simulink library "controls_element_lib"  (R2018b)
settings: Solver=VariableStepAuto  StartTime=0.0  StopTime=10.0  RelTol=1e-3
undefined symbols (not defined in the file): F_NOM, I_INV_BASE, j, P_INV_NOM, S_INV_NOM, S_NOM, S_PLANT, VHV_NOM, VLL_INV_NOM, VLL_NOM, Z_INV_BASE
libraries: simulink x20, $bdroot x5
(part 1 of 2)
settings Model: Creator=HussamAlatrash  LastModifiedBy=ahhei
settings DataIOCC: ReturnWorkspaceOutputs=on
settings DebuggingCC: UnconnectedInputMsg=none  UnconnectedOutputMsg=none  UnconnectedLineMsg=none
settings ModelReferenceCC: EnableRefExpFcnMdlSchedulingChecks=off
settings RTWCC: Description=Generic Real-Time Target
settings ConfigComp: CovBoundaryAbsTol=1.0e-5

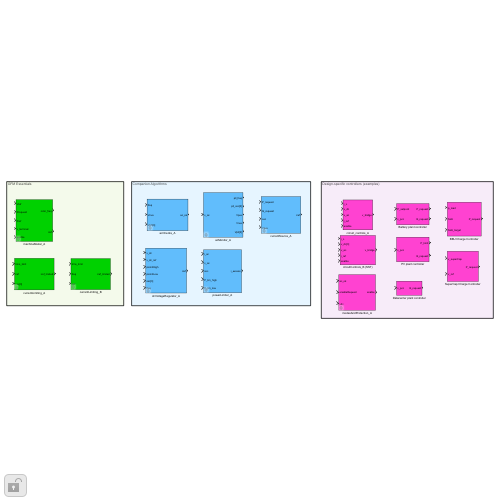
[thumbnail: Simulink's stored preview of the top-level diagram]
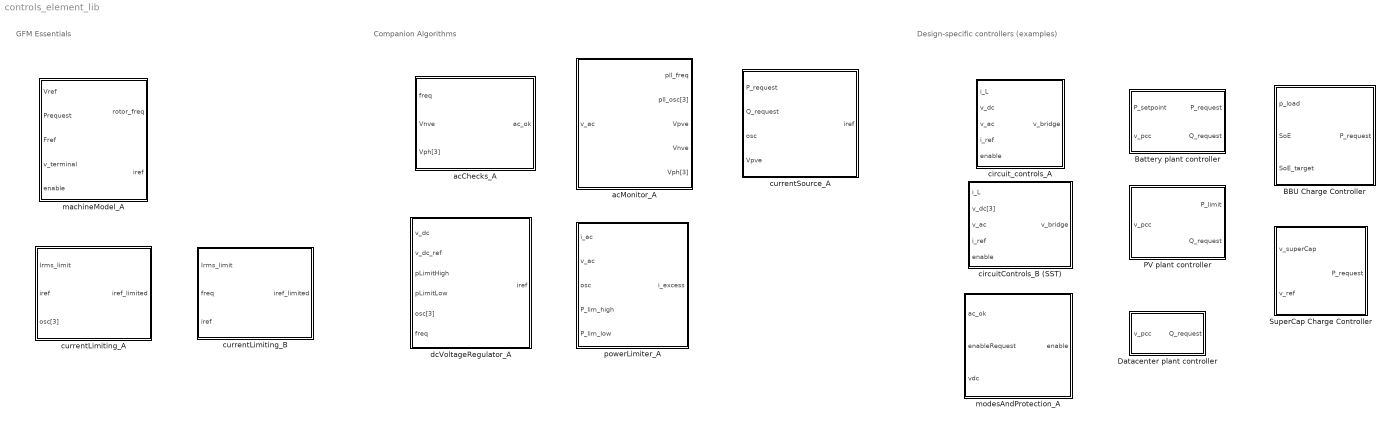
== system controls_element_lib ==
  note: Design-specific controllers (examples)
  note: Companion Algorithms
  note: GFM Essentials
  BBU Charge Controller : Subsystem
  Battery plant controller : Subsystem
  Datacenter plant controller : Subsystem
  PV plant controller : Subsystem
  SuperCap Charge Controller : Subsystem
  acChecks_A : Subsystem  mask{VllRated=VLL_NOM, nominalFrequency=F_NOM, tRequalify=2, T_CNTL=1e-3}
      mask prompts: VllRated "Rated line-to-line voltage (V)"; nominalFrequency "Nominal line frequency (Hz)"; tRequalify "Reconnection time (sec)"; T_CNTL "Operating sample time"
  acMonitor_A : Subsystem  mask{VllRated=VLL_NOM, nominalFrequency=F_NOM}
      mask prompts: VllRated "Rated line-to-line voltage (V)"; nominalFrequency "Nominal line frequency (Hz)"
  circuitControls_B (SST) : Subsystem
  circuit_controls_A : Subsystem
  currentLimiting_A : Subsystem  mask{IRated=I_INV_BASE, peakSoftLimit=2.6, peakHardLimit=3.6}
      mask prompts: IRated "Rated current (A)"; peakSoftLimit "Soft peak limit (pu)"; peakHardLimit "Hard peak limit (pu)"
  currentLimiting_B : Subsystem  mask{IRated=I_INV_BASE, peakSoftLimit=2.6, peakHardLimit=3.6}
      mask prompts: IRated "Rated current (A)"; peakSoftLimit "Soft peak limit (pu)"; peakHardLimit "Hard peak limit (pu)"
  currentSource_A : Subsystem  mask{VllRated=VLL_NOM, SRated=S_NOM, nominalFrequency=F_NOM, Plimit=1, Qlimit=0.43}
      mask prompts: VllRated "Rated line-to-line voltage (V)"; SRated "Rated power (VA)"; nominalFrequency "Nominal line frequency (Hz)"; Plimit "Real power request limit (pu)"; Qlimit "Reactive power request limit (pu)"
  dcVoltageRegulator_A : Subsystem  mask{kp=20e3, kSlowPath=0, wSlowPath=5, pLimitExternalMinimum=0.05*S_NOM, vdc_deadband=0, VllRated=VLL_INV_NOM}
      mask prompts: kp "Proportional gain (W/V)"; kSlowPath "Slow path gain (W/V)"; wSlowPath "Slow path bandwidth (rad)"; pLimitExternalMinimum "Minimum value for external power limit (W)"; vdc_deadband "Deadband around reference voltage (V)"; VllRated "Rated Voltage (Volts, line-to-line)"
  machineModel_A : Subsystem  mask{SRated=S_INV_NOM, VllRated=VLL_INV_NOM, nominalFrequency=F_NOM, inertialConstant=2.5, kDroop=1, kDamper=2, Xs=0.3, rs=0.08, Qlimit=0.5, wExciter=10}
      mask prompts: SRated "Rated power (VA)"; VllRated "Rated Voltage (Volts, line-to-line)"; nominalFrequency "Nominal frequency (Hz)"; inertialConstant "Inertial constant (seconds)"; kDroop "Droop gain (pu/Hz)"; kDamper "Damper gain (pu/Hz)"; Xs "Stator reactance (pu)"; rs "Stator resistance (pu)"; Qlimit "Reactive power request limit (pu)"; wExciter "Exciter Bandwidth (rad)"
  modesAndProtection_A : Subsystem  mask{dcOvervotlageThreshold=1800, dcUndervotlageThreshold=700, dcTripClearTimeout=0.2}
      mask prompts: dcOvervotlageThreshold "Dc overvoltage threshold"; dcUndervotlageThreshold "Dc undervoltage threshold"; dcTripClearTimeout "Dc protection clear time"
  powerLimiter_A : Subsystem  mask{VllRated=VLL_NOM, nominalFrequency=F_NOM, wPowerLimiter=3}
      mask prompts: VllRated "Rated line-to-line voltage (V)"; nominalFrequency "Nominal line frequency (Hz)"; wPowerLimiter "Bandwidth (rad)"

== system controls_element_lib/BBU Charge Controller ==
  p_load : Inport
  SoE : Inport  Port=2
  SoE_target : Inport  Port=3
  Gain : Gain  Gain=-1
  Gain4 : Gain  Gain=1e6/0.25
  Saturation1 : Saturate  UpperLimit=P_INV_NOM  LowerLimit=-P_INV_NOM
  Sum2 : Sum  Inputs=++|
  Sum3 : Sum  Inputs=|+-
  Transfer Fcn : TransferFcn  Denominator=[0.2 1]
  Transfer Fcn1 : TransferFcn  Denominator=[5 1]
  P_request : Outport
  wires:
  SoE/1 -> Sum3/1
  Gain/1 -> Transfer Fcn1/1
  Saturation1/1 -> Sum2/2  "P_charge_control"
  Sum3/1 -> Transfer Fcn/1
  SoE_target/1 -> Sum3/2
  Transfer Fcn1/1 -> Sum2/1  "P_dc"
  Gain4/1 -> Saturation1/1
  Sum2/1 -> P_request/1
  p_load/1 -> Gain/1
  Transfer Fcn/1 -> Gain4/1

== system controls_element_lib/Battery plant controller ==
  P_setpoint : Inport
  v_pcc : Inport  Port=2
  Gain : Gain  Gain=-1
  Gain1 : Gain  Gain=S_PLANT
  Gain2 : Gain  Gain=S_PLANT
  Gain4 : Gain  Gain=1/VHV_NOM
  LVRT_foldback : Subsystem
  Meter : Subsystem
  Saturation : Saturate  UpperLimit=0.9*S_PLANT  LowerLimit=-0.9*S_PLANT
  Saturation Dynamic : simulink/Discontinuities/Saturation Dynamic  OutMin=[]  OutMax=[]  OutDataTypeStr=Inherit: Same as second input  OutDataType=fixdt(1, 16)  OutScaling=2^-10  DoSatur=off
  VoltVAr : Subsystem
  P_request : Outport
  Q_request : Outport  Port=2
  wires:
  VoltVAr/1(Q) -> Gain1/1
  Meter/1(V_estimate) -> LVRT_foldback/1(Vpve_pu), VoltVAr/1(V)  "V_pu_plant"
  Gain1/1 -> Q_request/1  "Q_request"
  v_pcc/1 -> Gain4/1
  P_setpoint/1 -> Saturation/1
  Gain4/1 -> Meter/1(v)
  Saturation/1 -> Saturation Dynamic/2
  Gain2/1 -> Gain/1, Saturation Dynamic/1
  LVRT_foldback/1(limit_pu) -> Gain2/1  "spinout_limit_Vpcc"
  Saturation Dynamic/1 -> P_request/1  "P_request"
  Gain/1 -> Saturation Dynamic/3

== system controls_element_lib/Datacenter plant controller ==
  v_pcc : Inport
  Gain4 : Gain  Gain=1/VLL_INV_NOM
  Meter : Subsystem
  SRated2 : Gain  Gain=S_PLANT
  VoltVAr : Subsystem
  Q_request : Outport
  wires:
  VoltVAr/1(Q) -> SRated2/1
  Gain4/1 -> Meter/1(v)
  Meter/1(V_estimate) -> VoltVAr/1(V)  "V_pu_plant"
  SRated2/1 -> Q_request/1  "Q_request"
  v_pcc/1 -> Gain4/1

== system controls_element_lib/PV plant controller ==
  v_pcc : Inport
  Frequency foldback : Subsystem
  Gain1 : Gain  Gain=S_PLANT
  Gain2 : Gain  Gain=S_PLANT
  Gain4 : Gain  Gain=1/VHV_NOM
  Meter : Subsystem
  VoltVAr : Subsystem
  P_limit : Outport
  Q_request : Outport  Port=2
  wires:
  VoltVAr/1(Q) -> Gain1/1
  Gain4/1 -> Meter/1(v)
  Meter/2(V_estimate) -> VoltVAr/1(V)  "V_pu_plant"
  Gain1/1 -> Q_request/1  "Q_request"
  v_pcc/1 -> Gain4/1
  Meter/1(f) -> Frequency foldback/1(f)
  Frequency foldback/1(limit_pu) -> Gain2/1
  Gain2/1 -> P_limit/1  "P_limit"

== system controls_element_lib/SuperCap Charge Controller ==
  v_superCap : Inport
  v_ref : Inport  Port=2
  Gain4 : Gain  Gain=S_INV_NOM/100
  Saturation1 : Saturate  UpperLimit=S_INV_NOM  LowerLimit=-S_INV_NOM
  Sum3 : Sum  Inputs=|+-
  P_request : Outport
  wires:
  Saturation1/1 -> P_request/1
  v_ref/1 -> Sum3/2
  Sum3/1 -> Gain4/1
  v_superCap/1 -> Sum3/1
  Gain4/1 -> Saturation1/1

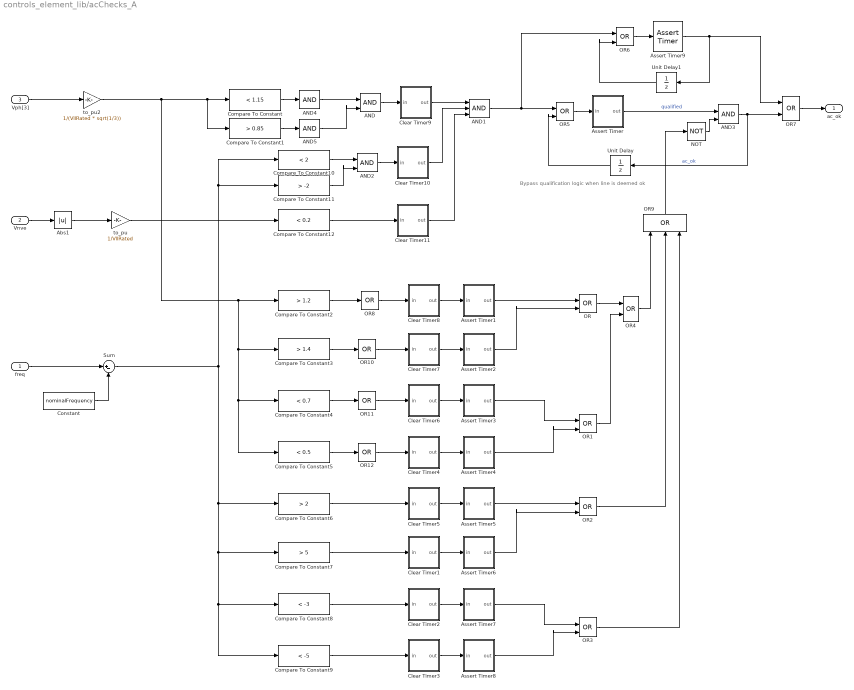
== system controls_element_lib/acChecks_A ==
  note: Bypass qualification logic when line is deemed ok
  freq : Inport
  Vnve : Inport  Port=2
  Vph[3] : Inport  Port=3
  AND : Logic  IconShape=distinctive  AllPortsSameDT=off  OutDataTypeStr=boolean
  AND1 : Logic  Inputs=3  IconShape=distinctive  AllPortsSameDT=off  OutDataTypeStr=boolean
  AND2 : Logic  IconShape=distinctive  AllPortsSameDT=off  OutDataTypeStr=boolean
  AND3 : Logic  IconShape=distinctive  AllPortsSameDT=off  OutDataTypeStr=boolean
  AND4 : Logic  Inputs=1  IconShape=distinctive  AllPortsSameDT=off  OutDataTypeStr=boolean
  AND5 : Logic  Inputs=1  IconShape=distinctive  AllPortsSameDT=off  OutDataTypeStr=boolean
  Abs1 : Abs
  Assert Timer : Subsystem  mask{T_STEP=T_CNTL, TIMEOUT=300}
      mask prompts: T_STEP "Time step"
  Assert Timer1 : Subsystem  mask{T_STEP=T_CNTL, TIMEOUT=60}
      mask prompts: T_STEP "Time step"
  Assert Timer2 : Subsystem  mask{T_STEP=T_CNTL, TIMEOUT=10}
      mask prompts: T_STEP "Time step"
  Assert Timer3 : Subsystem  mask{T_STEP=T_CNTL, TIMEOUT=60}
      mask prompts: T_STEP "Time step"
  Assert Timer4 : Subsystem  mask{T_STEP=T_CNTL, TIMEOUT=10}
      mask prompts: T_STEP "Time step"
  Assert Timer5 : Subsystem  mask{T_STEP=T_CNTL, TIMEOUT=60}
      mask prompts: T_STEP "Time step"
  Assert Timer6 : Subsystem  mask{T_STEP=T_CNTL, TIMEOUT=10}
      mask prompts: T_STEP "Time step"
  Assert Timer7 : Subsystem  mask{T_STEP=T_CNTL, TIMEOUT=60}
      mask prompts: T_STEP "Time step"
  Assert Timer8 : Subsystem  mask{T_STEP=T_CNTL, TIMEOUT=10}
      mask prompts: T_STEP "Time step"
  Assert Timer9 : $bdroot/acChecks_A/Assert Timer  T_STEP=T_CNTL  TIMEOUT=tRequalify
  Clear Timer1 : Subsystem  mask{T_STEP=T_CNTL, TIMEOUT=0.1, TIMER_INIT=0.1}
      mask prompts: T_STEP "Time step"; TIMER_INIT "Timer initial value"
  Clear Timer10 : Subsystem  mask{T_STEP=T_CNTL, TIMEOUT=0.1, TIMER_INIT=0}
      mask prompts: T_STEP "Time step"; TIMER_INIT "Timer initial value"
  Clear Timer11 : Subsystem  mask{T_STEP=T_CNTL, TIMEOUT=0.1, TIMER_INIT=0}
      mask prompts: T_STEP "Time step"; TIMER_INIT "Timer initial value"
  Clear Timer2 : Subsystem  mask{T_STEP=T_CNTL, TIMEOUT=0.1, TIMER_INIT=0.1}
      mask prompts: T_STEP "Time step"; TIMER_INIT "Timer initial value"
  Clear Timer3 : Subsystem  mask{T_STEP=T_CNTL, TIMEOUT=0.1, TIMER_INIT=0.1}
      mask prompts: T_STEP "Time step"; TIMER_INIT "Timer initial value"
  Clear Timer4 : Subsystem  mask{T_STEP=T_CNTL, TIMEOUT=0.1, TIMER_INIT=0}
      mask prompts: T_STEP "Time step"; TIMER_INIT "Timer initial value"
  Clear Timer5 : Subsystem  mask{T_STEP=T_CNTL, TIMEOUT=0.1, TIMER_INIT=0.1}
      mask prompts: T_STEP "Time step"; TIMER_INIT "Timer initial value"
  Clear Timer6 : Subsystem  mask{T_STEP=T_CNTL, TIMEOUT=0.1, TIMER_INIT=0}
      mask prompts: T_STEP "Time step"; TIMER_INIT "Timer initial value"
  Clear Timer7 : Subsystem  mask{T_STEP=T_CNTL, TIMEOUT=0.1, TIMER_INIT=0}
      mask prompts: T_STEP "Time step"; TIMER_INIT "Timer initial value"
  Clear Timer8 : Subsystem  mask{T_STEP=T_CNTL, TIMEOUT=0.1, TIMER_INIT=0}
      mask prompts: T_STEP "Time step"; TIMER_INIT "Timer initial value"
  Clear Timer9 : Subsystem  mask{T_STEP=T_CNTL, TIMEOUT=0.1, TIMER_INIT=0}
      mask prompts: T_STEP "Time step"; TIMER_INIT "Timer initial value"
  Compare To Constant : simulink/Logic and Bit Operations/Compare To Constant  relop=<  const=1.15  OutDataTypeStr=boolean
  Compare To Constant1 : simulink/Logic and Bit Operations/Compare To Constant  relop=>  const=0.85  OutDataTypeStr=boolean
  Compare To Constant10 : simulink/Logic and Bit Operations/Compare To Constant  relop=<  const=2  OutDataTypeStr=boolean
  Compare To Constant11 : simulink/Logic and Bit Operations/Compare To Constant  relop=>  const=-2  OutDataTypeStr=boolean
  Compare To Constant12 : simulink/Logic and Bit Operations/Compare To Constant  relop=<  const=0.2  OutDataTypeStr=boolean
  Compare To Constant2 : simulink/Logic and Bit Operations/Compare To Constant  relop=>  const=1.2  OutDataTypeStr=boolean
  Compare To Constant3 : simulink/Logic and Bit Operations/Compare To Constant  relop=>  const=1.4  OutDataTypeStr=boolean
  Compare To Constant4 : simulink/Logic and Bit Operations/Compare To Constant  relop=<  const=0.7  OutDataTypeStr=boolean
  Compare To Constant5 : simulink/Logic and Bit Operations/Compare To Constant  relop=<  const=0.5  OutDataTypeStr=boolean
  Compare To Constant6 : simulink/Logic and Bit Operations/Compare To Constant  relop=>  const=2  OutDataTypeStr=boolean
  Compare To Constant7 : simulink/Logic and Bit Operations/Compare To Constant  relop=>  const=5  OutDataTypeStr=boolean
  Compare To Constant8 : simulink/Logic and Bit Operations/Compare To Constant  relop=<  const=-3  OutDataTypeStr=boolean
  Compare To Constant9 : simulink/Logic and Bit Operations/Compare To Constant  relop=<  const=-5  OutDataTypeStr=boolean
  Constant : Constant  Value=nominalFrequency
  NOT : Logic  Operator=NOT  IconShape=distinctive  AllPortsSameDT=off  OutDataTypeStr=boolean
  OR{,1..7} (8 alike) : Logic  Operator=OR  IconShape=distinctive  AllPortsSameDT=off  OutDataTypeStr=boolean
  OR{8,10..12} (4 alike) : Logic  Operator=OR  Inputs=1  IconShape=distinctive  AllPortsSameDT=off  OutDataTypeStr=boolean
  OR9 : Logic  Operator=OR  Inputs=3  IconShape=distinctive  AllPortsSameDT=off  OutDataTypeStr=boolean
  Sum : Sum  Inputs=|+-
  Unit Delay : UnitDelay  SampleTime=T_CNTL  HasFrameUpgradeWarning=on
  Unit Delay1 : UnitDelay  SampleTime=T_CNTL  HasFrameUpgradeWarning=on
  to_pu : Gain  Gain=1/VllRated
  to_pu2 : Gain  Gain=1/(VllRated * sqrt(1/3))
  ac_ok : Outport
  wires:
  AND5/1 -> AND/2
  AND4/1 -> AND/1
  AND/1 -> Clear Timer9/1(in)
  OR12/1 -> Clear Timer4/1(in)
  OR11/1 -> Clear Timer6/1(in)
  OR10/1 -> Clear Timer7/1(in)
  OR8/1 -> Clear Timer8/1(in)
  OR2/1 -> OR9/2
  AND3/1 -> OR7/2, Unit Delay/1  "ac_ok"
  Clear Timer4/1(out) -> Assert Timer4/1(in)
  OR/1 -> OR4/1
  Clear Timer9/1(out) -> AND1/1
  Compare To Constant10/1 -> AND2/1
  Assert Timer2/1(out) -> OR/2
  Sum/1 -> Compare To Constant9/1, Compare To Constant8/1, Compare To Constant7/1, Compare To Constant6/1, Compare To Constant10/1, Compare To Constant11/1
  Clear Timer7/1(out) -> Assert Timer2/1(in)
  Clear Timer3/1(out) -> Assert Timer8/1(in)
  Clear Timer10/1(out) -> AND1/2
  Compare To Constant7/1 -> Clear Timer1/1(in)
  Compare To Constant5/1 -> OR12/1
  Clear Timer2/1(out) -> Assert Timer7/1(in)
  OR1/1 -> OR4/2
  Compare To Constant8/1 -> Clear Timer2/1(in)
  AND1/1 -> OR5/1, OR6/1
  Clear Timer6/1(out) -> Assert Timer3/1(in)
  Assert Timer6/1(out) -> OR2/2
  Compare To Constant4/1 -> OR11/1
  Compare To Constant11/1 -> AND2/2
  Compare To Constant9/1 -> Clear Timer3/1(in)
  AND2/1 -> Clear Timer10/1(in)
  Compare To Constant3/1 -> OR10/1
  Compare To Constant/1 -> AND4/1
  Assert Timer3/1(out) -> OR1/1
  NOT/1 -> AND3/2
  Vnve/1 -> Abs1/1
  Assert Timer8/1(out) -> OR3/2
  Assert Timer7/1(out) -> OR3/1
  Clear Timer8/1(out) -> Assert Timer1/1(in)
  Clear Timer1/1(out) -> Assert Timer6/1(in)
  Compare To Constant6/1 -> Clear Timer5/1(in)
  Clear Timer5/1(out) -> Assert Timer5/1(in)
  Assert Timer5/1(out) -> OR2/1
  Assert Timer4/1(out) -> OR1/2
  OR3/1 -> OR9/3
  Assert Timer/1(out) -> AND3/1  "qualified"
  Compare To Constant1/1 -> AND5/1
  Compare To Constant2/1 -> OR8/1
  OR5/1 -> Assert Timer/1(in)
  Clear Timer11/1(out) -> AND1/3
  Compare To Constant12/1 -> Clear Timer11/1(in)
  Assert Timer1/1(out) -> OR/1
  Unit Delay/1 -> OR5/2
  Abs1/1 -> to_pu/1
  to_pu2/1 -> Compare To Constant3/1, Compare To Constant4/1, Compare To Constant5/1, Compare To Constant2/1, Compare To Constant1/1, Compare To Constant/1
  to_pu/1 -> Compare To Constant12/1
  freq/1 -> Sum/1
  Constant/1 -> Sum/2
  Unit Delay1/1 -> OR6/2
  OR6/1 -> Assert Timer9/1
  Assert Timer9/1 -> OR7/1, Unit Delay1/1
  OR7/1 -> ac_ok/1
  OR9/1 -> NOT/1
  OR4/1 -> OR9/1
  Vph[3]/1 -> to_pu2/1

== system controls_element_lib/acMonitor_A ==
  v_ac : Inport
  Analyzer_V : Subsystem
  Gain2 : Gain  Gain=2
  PLL_3ph : Subsystem
  RMS_Analyzer : Subsystem
  SOGI : Subsystem
  to_pu : Gain  Gain=1/VllRated
  pll_freq : Outport
  pll_osc[3] : Outport  Port=2
  Vpve : Outport  Port=3
  Vnve : Outport  Port=4
  Vph[3] : Outport  Port=5
  wires:
  to_pu/1 -> PLL_3ph/1(ref)
  v_ac/1 -> RMS_Analyzer/1(in), Analyzer_V/1(in[3]), to_pu/1
  PLL_3ph/2(freq) -> pll_freq/1, Gain2/1
  PLL_3ph/1(osc[3]) -> Analyzer_V/2(osc[3]), pll_osc[3]/1
  Analyzer_V/3(Pve) -> Vpve/1
  Analyzer_V/4(Nve) -> Vnve/1
  RMS_Analyzer/1(RMS) -> SOGI/1(in)
  Gain2/1 -> SOGI/2(fnom)
  SOGI/1(notch) -> Vph[3]/1

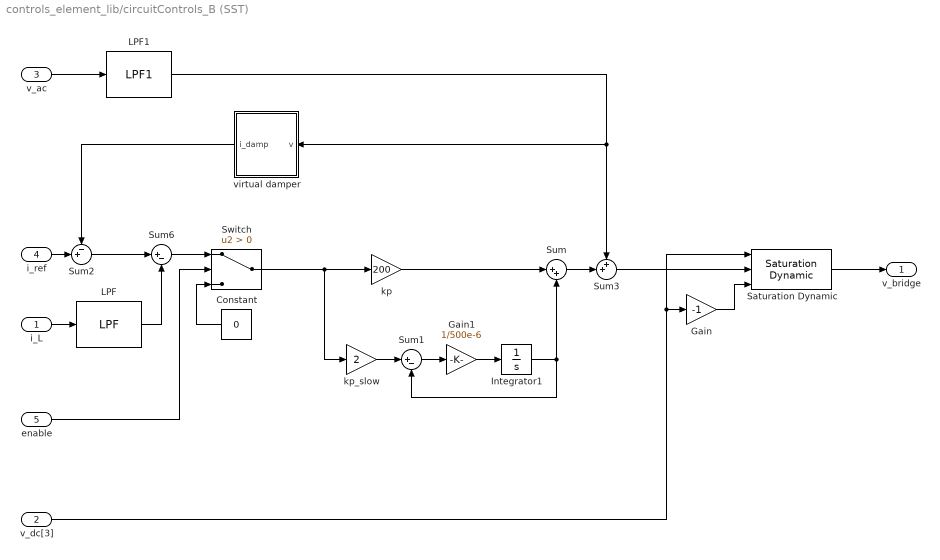
== system controls_element_lib/circuitControls_B (SST) ==
  i_L : Inport
  v_dc[3] : Inport  Port=2
  v_ac : Inport  Port=3
  i_ref : Inport  Port=4
  enable : Inport  Port=5
  Constant : Constant  Value=0
  Gain : Gain  Gain=-1
  Gain1 : Gain  Gain=1/500e-6
  Integrator1 : Integrator
  LPF : $bdroot/circuit_controls_A/LPF  SystemSampleTime=-1  EmptyChoice=off  PassThrough=off  PassThroughVariantControl=(default)  EmptyChoiceVariantControl=(default)  Latency=0  AutoFrameSizeCalculation=off
  LPF1 : $bdroot/circuit_controls_A/LPF1  SystemSampleTime=-1  EmptyChoice=off  PassThrough=off  PassThroughVariantControl=(default)  EmptyChoiceVariantControl=(default)  Latency=0  AutoFrameSizeCalculation=off
  Saturation Dynamic : simulink/Discontinuities/Saturation Dynamic  OutMin=[]  OutMax=[]  OutDataTypeStr=Inherit: Same as second input  OutDataType=fixdt(1, 16)  OutScaling=2^-10  DoSatur=off
  Sum : Sum  Inputs=|++
  Sum1 : Sum  Inputs=|+-
  Sum2 : Sum  Inputs=-+|
  Sum3 : Sum  Inputs=++|
  Sum6 : Sum  Inputs=|+-
  Switch : Switch  Criteria=u2 > Threshold
  kp : Gain  Gain=200
  kp_slow : Gain  Gain=2
  virtual damper : Subsystem
  v_bridge : Outport
  wires:
  Gain/1 -> Saturation Dynamic/3
  kp_slow/1 -> Sum1/1
  Gain1/1 -> Integrator1/1
  Sum1/1 -> Gain1/1
  Integrator1/1 -> Sum1/2, Sum/2
  kp/1 -> Sum/1
  Sum2/1 -> Sum6/1
  Saturation Dynamic/1 -> v_bridge/1
  i_L/1 -> LPF/1
  Switch/1 -> kp/1, kp_slow/1
  i_ref/1 -> Sum2/2
  virtual damper/1(i_damp) -> Sum2/1
  v_ac/1 -> LPF1/1
  Sum3/1 -> Saturation Dynamic/2
  v_dc[3]/1 -> Saturation Dynamic/1, Gain/1
  enable/1 -> Switch/2
  Constant/1 -> Switch/3
  LPF/1 -> Sum6/2
  Sum6/1 -> Switch/1
  Sum/1 -> Sum3/2
  LPF1/1 -> virtual damper/1(v), Sum3/1

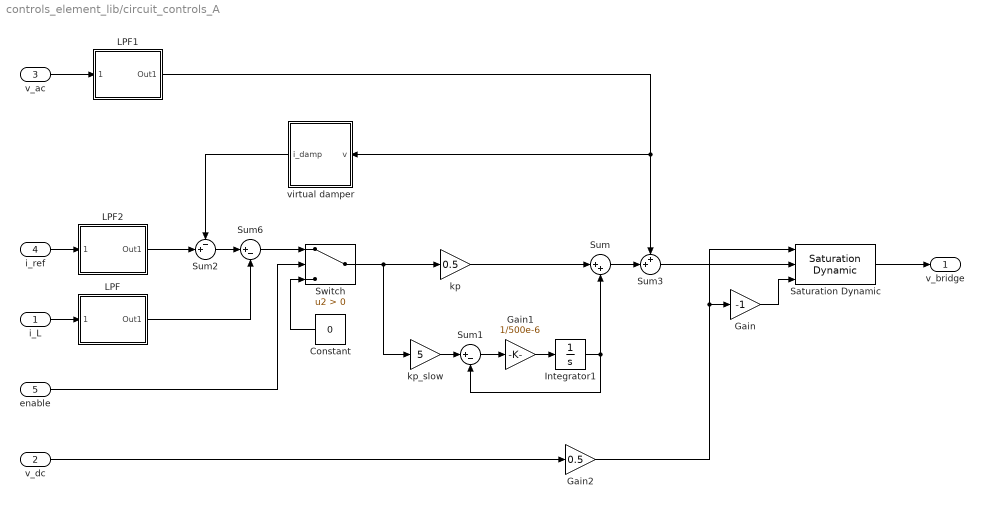
== system controls_element_lib/circuit_controls_A ==
  i_L : Inport
  v_dc : Inport  Port=2
  v_ac : Inport  Port=3
  i_ref : Inport  Port=4
  enable : Inport  Port=5
  Constant : Constant  Value=0
  Gain : Gain  Gain=-1
  Gain1 : Gain  Gain=1/500e-6
  Gain2 : Gain  Gain=0.5
  Integrator1 : Integrator
  LPF : Subsystem
  LPF1 : Subsystem
  LPF2 : Subsystem
  Saturation Dynamic : simulink/Discontinuities/Saturation Dynamic  OutMin=[]  OutMax=[]  OutDataTypeStr=Inherit: Same as second input  OutDataType=fixdt(1, 16)  OutScaling=2^-10  DoSatur=off
  Sum : Sum  Inputs=|++
  Sum1 : Sum  Inputs=|+-
  Sum2 : Sum  Inputs=-+|
  Sum3 : Sum  Inputs=++|
  Sum6 : Sum  Inputs=|+-
  Switch : Switch  Criteria=u2 > Threshold
  kp : Gain  Gain=0.5
  kp_slow : Gain  Gain=5
  virtual damper : Subsystem
  v_bridge : Outport
  wires:
  LPF2/1(Out1) -> Sum2/2
  Gain/1 -> Saturation Dynamic/3
  v_dc/1 -> Gain2/1
  kp_slow/1 -> Sum1/1
  Gain1/1 -> Integrator1/1
  Sum1/1 -> Gain1/1
  Integrator1/1 -> Sum1/2, Sum/2
  kp/1 -> Sum/1
  Sum2/1 -> Sum6/1
  Sum/1 -> Sum3/2
  Saturation Dynamic/1 -> v_bridge/1
  i_L/1 -> LPF/1(1)
  Switch/1 -> kp_slow/1, kp/1
  i_ref/1 -> LPF2/1(1)
  virtual damper/1(i_damp) -> Sum2/1
  Sum3/1 -> Saturation Dynamic/2
  Sum6/1 -> Switch/1
  Constant/1 -> Switch/3
  enable/1 -> Switch/2
  v_ac/1 -> LPF1/1(1)
  Gain2/1 -> Saturation Dynamic/1, Gain/1
  LPF/1(Out1) -> Sum6/2
  LPF1/1(Out1) -> virtual damper/1(v), Sum3/1

== system controls_element_lib/currentLimiting_A ==
  Irms_limit : Inport
  iref : Inport  Port=2
  osc[3] : Inport  Port=3
  Analyzer_I : Subsystem
  Sum2 : Sum  Inputs=|+-
  excess_sink : Subsystem
  soft_saturation : Subsystem  mask{soft_limit=peakSoftLimit*IRated, hard_limit=peakHardLimit*IRated}
      mask prompts: soft_limit "Soft limit"; hard_limit "Hard limit"
  iref_limited : Outport
  wires:
  Sum2/1 -> soft_saturation/1(in)
  osc[3]/1 -> Analyzer_I/2(osc[3]), excess_sink/2(osc[3])
  iref/1 -> Sum2/1, Analyzer_I/1(in[3])
  excess_sink/1(i_excess[3]) -> Sum2/2
  Analyzer_I/1(fund[3]) -> excess_sink/1(I_total[3])  "I_total[3]"
  soft_saturation/1(out) -> iref_limited/1
  Irms_limit/1 -> excess_sink/3(Irms_limit)

== system controls_element_lib/currentLimiting_B ==
  Irms_limit : Inport
  freq : Inport  Port=2
  iref : Inport  Port=3
  Product1 : Product
  RMS_Analyzer : Subsystem
  SOGI_BPF : Subsystem
  Sum1 : Sum  Inputs=|+-
  estimate_excess : Subsystem
  soft_saturation : Subsystem  mask{soft_limit=peakSoftLimit*IRated, hard_limit=peakHardLimit*IRated}
      mask prompts: soft_limit "Soft limit"; hard_limit "Hard limit"
  iref_limited : Outport
  wires:
  Irms_limit/1 -> estimate_excess/1(Ilimit)
  iref/1 -> SOGI_BPF/1(in), RMS_Analyzer/1(in), Sum1/1
  freq/1 -> SOGI_BPF/2(f)
  SOGI_BPF/1(bpf) -> Product1/2
  Sum1/1 -> soft_saturation/1(in)
  Product1/1 -> Sum1/2  "i_excess"
  RMS_Analyzer/1(RMS) -> estimate_excess/2(I[3])  "Irms"
  estimate_excess/1(excess_fraction) -> Product1/1
  soft_saturation/1(out) -> iref_limited/1

== system controls_element_lib/currentSource_A ==
  note: Positive Q requires negative Iq
  P_request : Inport
  Q_request : Inport  Port=2
  osc : Inport  Port=3
  Vpve : Inport  Port=4
  Complex to Real-Imag : ComplexToRealImag
  Conj : Math  Operator=conj  SaturateOnIntegerOverflow=on
  Divide : Product  Inputs=*/
  Gain : Gain  Gain=1/sqrt(3)
  Max1 : MinMax  Function=max  Inputs=2
  Real-Imag to Complex : RealImagToComplex
  VLL_RATED : Constant  Value=VllRated
  current_modulator : Subsystem
  iref : Outport
  wires:
  Gain/1 -> current_modulator/1(I_cmd)
  Conj/1 -> Divide/1
  Real-Imag to Complex/1 -> Conj/1
  osc/1 -> current_modulator/2(osc)
  current_modulator/1(i_ref) -> iref/1
  Vpve/1 -> Complex to Real-Imag/1
  Divide/1 -> Gain/1
  Max1/1 -> Divide/2
  VLL_RATED/1 -> Max1/2
  Complex to Real-Imag/1 -> Max1/1
  P_request/1 -> Real-Imag to Complex/1
  Q_request/1 -> Real-Imag to Complex/2

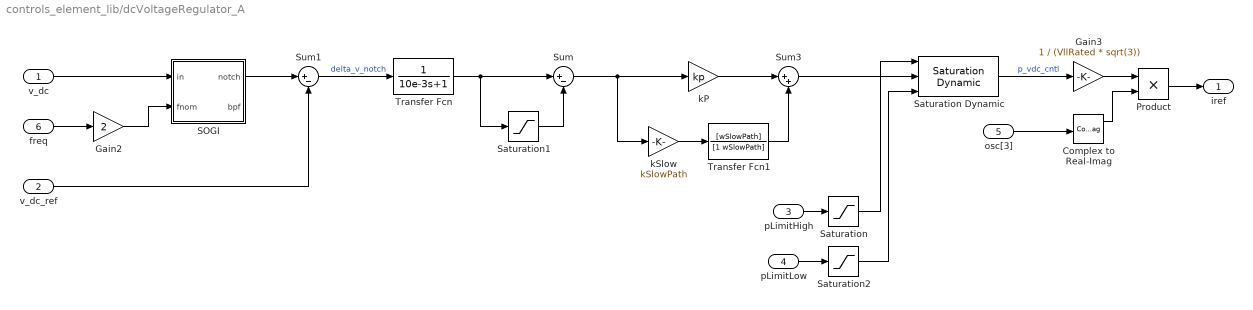
== system controls_element_lib/dcVoltageRegulator_A ==
  v_dc : Inport
  v_dc_ref : Inport  Port=2
  pLimitHigh : Inport  Port=3
  pLimitLow : Inport  Port=4
  osc[3] : Inport  Port=5
  freq : Inport  Port=6
  Complex to Real-Imag : ComplexToRealImag
  Gain2 : Gain  Gain=2
  Gain3 : Gain  Gain=1 / (VllRated * sqrt(3))
  Product : Product
  SOGI : Subsystem
  Saturation : Saturate  UpperLimit=inf  LowerLimit=pLimitExternalMinimum
  Saturation Dynamic : simulink/Discontinuities/Saturation Dynamic  OutMin=[]  OutMax=[]  OutDataTypeStr=Inherit: Same as second input  OutDataType=fixdt(1, 16)  OutScaling=2^-10  DoSatur=off
  Saturation1 : Saturate  UpperLimit=vdc_deadband  LowerLimit=-vdc_deadband
  Saturation2 : Saturate  UpperLimit=-pLimitExternalMinimum  LowerLimit=-inf
  Sum : Sum  Inputs=|+-
  Sum1 : Sum  Inputs=|+-
  Sum3 : Sum  Inputs=|++
  Transfer Fcn : TransferFcn  Denominator=[10e-3 1]
  Transfer Fcn1 : TransferFcn  Numerator=[wSlowPath]  Denominator=[1 wSlowPath]
  kP : Gain  Gain=kp
  kSlow : Gain  Gain=kSlowPath
  iref : Outport
  wires:
  Saturation2/1 -> Saturation Dynamic/3
  Saturation/1 -> Saturation Dynamic/1
  kSlow/1 -> Transfer Fcn1/1
  Sum3/1 -> Saturation Dynamic/2
  kP/1 -> Sum3/1
  Sum/1 -> kSlow/1, kP/1
  Sum1/1 -> Transfer Fcn/1  "delta_v_notch"
  v_dc_ref/1 -> Sum1/2
  Saturation Dynamic/1 -> Gain3/1  "p_vdc_cntl"
  Transfer Fcn/1 -> Sum/1, Saturation1/1
  SOGI/1(notch) -> Sum1/1
  v_dc/1 -> SOGI/1(in)
  freq/1 -> Gain2/1
  Gain2/1 -> SOGI/2(fnom)
  Complex to Real-Imag/1 -> Product/2
  Gain3/1 -> Product/1
  Product/1 -> iref/1
  osc[3]/1 -> Complex to Real-Imag/1
  Saturation1/1 -> Sum/2
  Transfer Fcn1/1 -> Sum3/2
  pLimitLow/1 -> Saturation2/1
  pLimitHigh/1 -> Saturation/1

== system controls_element_lib/machineModel_A ==
  Vref : Inport
  Prequest : Inport  Port=2
  Fref : Inport  Port=3
  v_terminal : Inport  Port=4
  enable : Inport  Port=5
  excitation : Subsystem
  governer : Subsystem
  impedance emulation : Subsystem
  power analyzer : Subsystem
  rotor model : Subsystem
  voltage analyzer : Subsystem
  rotor_freq : Outport
  iref : Outport  Port=2
  wires:
  rotor model/1(osc[3]) -> excitation/2(osc[3]), voltage analyzer/1(osc[3])
  power analyzer/1(P) -> rotor model/2(p_electrical)  "p_electrical"
  excitation/1(v_emf) -> impedance emulation/1(v_emf)  "v_emf"
  governer/1(power) -> rotor model/1(p_mechanical)
  Prequest/1 -> governer/1(Prequest)
  impedance emulation/1(i_ref) -> power analyzer/1(iac), iref/1
  v_terminal/1 -> impedance emulation/3(v_terminal), power analyzer/2(vac), voltage analyzer/2(v_terminal)
  voltage analyzer/2(Vq) -> governer/5(Vq)
  rotor model/2(f_rotor) -> governer/6(f_rotor), rotor_freq/1  "f_rotor"
  voltage analyzer/1(Vd) -> excitation/3(Vd), governer/4(Vd)
  enable/1 -> impedance emulation/2(enable), governer/3(enabled)
  Fref/1 -> governer/2(Fref)
  Vref/1 -> excitation/1(VRef)

== system controls_element_lib/modesAndProtection_A ==
  ac_ok : Inport
  enableRequest : Inport  Port=2
  vdc : Inport  Port=3
  AND : Logic  Inputs=3  IconShape=distinctive  AllPortsSameDT=off  OutDataTypeStr=boolean
  hardware_protection : Subsystem
  enable : Outport
  wires:
  vdc/1 -> hardware_protection/1(vdc)
  hardware_protection/1(all_clear) -> AND/2  "protection_clear"
  enableRequest/1 -> AND/3
  AND/1 -> enable/1  "enable"
  ac_ok/1 -> AND/1

== system controls_element_lib/powerLimiter_A ==
  i_ac : Inport
  v_ac : Inport  Port=2
  osc : Inport  Port=3
  P_lim_high : Inport  Port=4
  P_lim_low : Inport  Port=5
  Gain1 : Gain  Gain=1/(VllRated * sqrt(3))
  Product : Product
  Saturation Dynamic : simulink/Discontinuities/Saturation Dynamic  OutMin=[]  OutMax=[]  OutDataTypeStr=Inherit: Same as second input  OutDataType=fixdt(1, 16)  OutScaling=2^-10  DoSatur=off
  Sum of Elements : Sum  Inputs=+
  Sum1 : Sum  Inputs=|+-
  Transfer Fcn : TransferFcn  Denominator=[1/wPowerLimiter, 1]
  current_modulator : $bdroot/currentSource_A/current_modulator  SystemSampleTime=-1  EmptyChoice=off  PassThrough=off  PassThroughVariantControl=(default)  EmptyChoiceVariantControl=(default)  Latency=0  AutoFrameSizeCalculation=off
  i_excess : Outport
  wires:
  v_ac/1 -> Product/2
  i_ac/1 -> Product/1
  Product/1 -> Sum of Elements/1
  osc/1 -> current_modulator/2
  Gain1/1 -> current_modulator/1
  Sum of Elements/1 -> Transfer Fcn/1  "P_inst"
  Sum1/1 -> Gain1/1
  P_lim_high/1 -> Saturation Dynamic/1
  P_lim_low/1 -> Saturation Dynamic/3
  Saturation Dynamic/1 -> Sum1/2
  current_modulator/1 -> i_excess/1
  Transfer Fcn/1 -> Saturation Dynamic/2, Sum1/1  "P_lpf"

== system controls_element_lib/Battery plant controller/LVRT_foldback ==
  Vpve_pu : Inport
  Complex to Magnitude-Angle : ComplexToMagnitudeAngle
  Constant1 : Constant
  Gain : Gain  Gain=5
  Saturation : Saturate  UpperLimit=1  LowerLimit=0.05
  Sum1 : Sum  Inputs=|+-
  Sum2 : Sum  Inputs=|++
  Transfer Fcn : TransferFcn  Denominator=[0.02 1]
  foldback_threshold : Constant  Value=0.8
  limit_pu : Outport
  wires:
  Saturation/1 -> limit_pu/1
  Vpve_pu/1 -> Complex to Magnitude-Angle/1
  foldback_threshold/1 -> Sum1/2
  Constant1/1 -> Sum2/2
  Sum2/1 -> Saturation/1
  Complex to Magnitude-Angle/1 -> Sum1/1
  Transfer Fcn/1 -> Gain/1
  Gain/1 -> Sum2/1
  Sum1/1 -> Transfer Fcn/1

== system controls_element_lib/Battery plant controller/Meter ==
  v : Inport
  Complex to Real-Imag : ComplexToRealImag
  Conj : Math  Operator=conj  SaturateOnIntegerOverflow=on
  Gain : Gain  Gain=sqrt(2)
  Gain1 : Gain  Gain=1/3
  Gain2 : Gain  Gain=sqrt(3)
  PLL-analog : Subsystem
  Product3 : Product
  Real-Imag to Complex : RealImagToComplex
  Sum of Elements1 : Sum  Inputs=+
  Transfer Fcn : TransferFcn  Denominator=[0.05 1]
  Transfer Fcn1 : TransferFcn  Denominator=[0.05 1]
  V_estimate : Outport
  wires:
  Transfer Fcn1/1 -> Real-Imag to Complex/2
  Sum of Elements1/1 -> Gain1/1
  Transfer Fcn/1 -> Real-Imag to Complex/1
  Product3/1 -> Sum of Elements1/1
  Complex to Real-Imag/2 -> Transfer Fcn1/1
  v/1 -> PLL-analog/1(ref), Product3/1
  Complex to Real-Imag/1 -> Transfer Fcn/1
  PLL-analog/2(osc) -> Conj/1
  Conj/1 -> Gain/1
  Real-Imag to Complex/1 -> Gain2/1
  Gain/1 -> Product3/2
  Gain1/1 -> Complex to Real-Imag/1
  Gain2/1 -> V_estimate/1

== system controls_element_lib/Battery plant controller/VoltVAr ==
  V : Inport
  Abs : Abs
  Constant1 : Constant
  Gain : Gain  Gain=6
  Saturation : Saturate
  Sum1 : Sum  Inputs=|+-
  Transfer Fcn : TransferFcn  Denominator=[0.05 1]
  Q : Outport
  wires:
  Gain/1 -> Saturation/1
  Sum1/1 -> Gain/1
  Constant1/1 -> Sum1/1
  Abs/1 -> Sum1/2
  V/1 -> Abs/1
  Saturation/1 -> Transfer Fcn/1
  Transfer Fcn/1 -> Q/1

== system controls_element_lib/Datacenter plant controller/Meter ==
  v : Inport
  Complex to Real-Imag : ComplexToRealImag
  Conj : Math  Operator=conj  SaturateOnIntegerOverflow=on
  Gain : Gain  Gain=sqrt(2)
  Gain1 : Gain  Gain=1/3
  Gain2 : Gain  Gain=sqrt(3)
  PLL-analog : Subsystem
  Product3 : Product
  Real-Imag to Complex : RealImagToComplex
  Sum of Elements1 : Sum  Inputs=+
  Transfer Fcn : TransferFcn  Denominator=[0.05 1]
  Transfer Fcn1 : TransferFcn  Denominator=[0.05 1]
  V_estimate : Outport
  wires:
  Transfer Fcn1/1 -> Real-Imag to Complex/2
  Sum of Elements1/1 -> Gain1/1
  Transfer Fcn/1 -> Real-Imag to Complex/1
  Product3/1 -> Sum of Elements1/1
  Complex to Real-Imag/2 -> Transfer Fcn1/1
  v/1 -> PLL-analog/1(ref), Product3/1
  Complex to Real-Imag/1 -> Transfer Fcn/1
  PLL-analog/2(osc) -> Conj/1
  Conj/1 -> Gain/1
  Real-Imag to Complex/1 -> Gain2/1
  Gain/1 -> Product3/2
  Gain1/1 -> Complex to Real-Imag/1
  Gain2/1 -> V_estimate/1

== system controls_element_lib/Datacenter plant controller/VoltVAr ==
  V : Inport
  Abs : Abs
  Complex to Real-Imag : ComplexToRealImag
  Constant1 : Constant
  Gain : Gain  Gain=6
  Saturation : Saturate
  Sum1 : Sum  Inputs=|+-
  Transfer Fcn : TransferFcn  Denominator=[0.05 1]
  Q : Outport
  wires:
  Gain/1 -> Saturation/1
  Sum1/1 -> Gain/1
  Constant1/1 -> Sum1/1
  Abs/1 -> Sum1/2
  V/1 -> Complex to Real-Imag/1, Abs/1
  Saturation/1 -> Transfer Fcn/1
  Transfer Fcn/1 -> Q/1
  Complex to Real-Imag/1 -> ?

== system controls_element_lib/PV plant controller/Frequency foldback ==
  f : Inport
  Constant : Constant  Value=F_NOM+0.5
  Gain : Gain  Gain=3
  Saturation : Saturate  UpperLimit=1  LowerLimit=0
  Sum : Sum  Inputs=|+-
  Transfer Fcn : TransferFcn  Denominator=[0.05 1]
  limit_pu : Outport
  wires:
  Sum/1 -> Transfer Fcn/1
  f/1 -> Sum/2
  Gain/1 -> Saturation/1
  Transfer Fcn/1 -> Gain/1
  Constant/1 -> Sum/1
  Saturation/1 -> limit_pu/1

== system controls_element_lib/PV plant controller/Meter ==
  v : Inport
  Complex to Real-Imag : ComplexToRealImag
  Conj : Math  Operator=conj  SaturateOnIntegerOverflow=on
  Gain : Gain  Gain=sqrt(2)
  Gain1 : Gain  Gain=1/3
  Gain2 : Gain  Gain=sqrt(3)
  PLL-analog : Subsystem
  Product3 : Product
  Real-Imag to Complex : RealImagToComplex
  Sum of Elements1 : Sum  Inputs=+
  Transfer Fcn : TransferFcn  Denominator=[0.005 1]
  Transfer Fcn1 : TransferFcn  Denominator=[0.005 1]
  f : Outport
  V_estimate : Outport  Port=2
  wires:
  Transfer Fcn1/1 -> Real-Imag to Complex/2
  Sum of Elements1/1 -> Gain1/1
  Transfer Fcn/1 -> Real-Imag to Complex/1
  Product3/1 -> Sum of Elements1/1
  Complex to Real-Imag/2 -> Transfer Fcn1/1
  v/1 -> PLL-analog/1(ref), Product3/1
  Complex to Real-Imag/1 -> Transfer Fcn/1
  PLL-analog/2(osc) -> Conj/1
  Conj/1 -> Gain/1
  Real-Imag to Complex/1 -> Gain2/1
  Gain/1 -> Product3/2
  Gain1/1 -> Complex to Real-Imag/1
  Gain2/1 -> V_estimate/1
  PLL-analog/1(freq) -> f/1  "pll_freq_pcc"

== system controls_element_lib/PV plant controller/VoltVAr ==
  V : Inport
  Abs : Abs
  Constant1 : Constant
  Gain : Gain  Gain=6
  Saturation : Saturate
  Sum1 : Sum  Inputs=|+-
  Transfer Fcn : TransferFcn  Denominator=[0.005 1]
  Q : Outport
  wires:
  Gain/1 -> Saturation/1
  Sum1/1 -> Gain/1
  Constant1/1 -> Sum1/1
  Abs/1 -> Sum1/2
  V/1 -> Abs/1
  Saturation/1 -> Transfer Fcn/1
  Transfer Fcn/1 -> Q/1

== system controls_element_lib/acChecks_A/Assert Timer ==
  in : Inport
  Constant : Constant  Value=T_STEP
  Constant1 : Constant  Value=0
  Constant2 : Constant  Value=TIMEOUT
  Min2 : MinMax  Inputs=2
  Relational Operator : RelationalOperator  Operator=>  OutDataTypeStr=boolean  RndMeth=Simplest
  Sum2 : Sum  Inputs=|++
  Switch : Switch  Criteria=u2 > Threshold
  Unit Delay : UnitDelay  SampleTime=T_STEP  HasFrameUpgradeWarning=on
  out : Outport
  wires:
  Sum2/1 -> Relational Operator/1, Min2/1
  Constant2/1 -> Min2/2, Relational Operator/2
  Constant/1 -> Sum2/1
  Min2/1 -> Switch/1
  Constant1/1 -> Switch/3
  Unit Delay/1 -> Sum2/2
  in/1 -> Switch/2
  Switch/1 -> Unit Delay/1
  Relational Operator/1 -> out/1

== system controls_element_lib/acChecks_A/Assert Timer1 ==
  in : Inport
  Constant : Constant  Value=T_STEP
  Constant1 : Constant  Value=0
  Constant2 : Constant  Value=TIMEOUT
  Min2 : MinMax  Inputs=2
  Relational Operator : RelationalOperator  Operator=>  OutDataTypeStr=boolean  RndMeth=Simplest
  Sum2 : Sum  Inputs=|++
  Switch : Switch  Criteria=u2 > Threshold
  Unit Delay : UnitDelay  SampleTime=T_STEP  HasFrameUpgradeWarning=on
  out : Outport
  wires:
  Relational Operator/1 -> out/1
  Switch/1 -> Unit Delay/1
  in/1 -> Switch/2
  Unit Delay/1 -> Sum2/2
  Constant1/1 -> Switch/3
  Min2/1 -> Switch/1
  Constant/1 -> Sum2/1
  Constant2/1 -> Relational Operator/2, Min2/2
  Sum2/1 -> Min2/1, Relational Operator/1

== system controls_element_lib/acChecks_A/Assert Timer2 ==
  in : Inport
  Constant : Constant  Value=T_STEP
  Constant1 : Constant  Value=0
  Constant2 : Constant  Value=TIMEOUT
  Min2 : MinMax  Inputs=2
  Relational Operator : RelationalOperator  Operator=>  OutDataTypeStr=boolean  RndMeth=Simplest
  Sum2 : Sum  Inputs=|++
  Switch : Switch  Criteria=u2 > Threshold
  Unit Delay : UnitDelay  SampleTime=T_STEP  HasFrameUpgradeWarning=on
  out : Outport
  wires:
  Sum2/1 -> Relational Operator/1, Min2/1
  Constant2/1 -> Min2/2, Relational Operator/2
  Constant/1 -> Sum2/1
  Min2/1 -> Switch/1
  Constant1/1 -> Switch/3
  Unit Delay/1 -> Sum2/2
  in/1 -> Switch/2
  Switch/1 -> Unit Delay/1
  Relational Operator/1 -> out/1

== system controls_element_lib/acChecks_A/Assert Timer3 ==
  in : Inport
  Constant : Constant  Value=T_STEP
  Constant1 : Constant  Value=0
  Constant2 : Constant  Value=TIMEOUT
  Min2 : MinMax  Inputs=2
  Relational Operator : RelationalOperator  Operator=>  OutDataTypeStr=boolean  RndMeth=Simplest
  Sum2 : Sum  Inputs=|++
  Switch : Switch  Criteria=u2 > Threshold
  Unit Delay : UnitDelay  SampleTime=T_STEP  HasFrameUpgradeWarning=on
  out : Outport
  wires:
  Relational Operator/1 -> out/1
  Switch/1 -> Unit Delay/1
  in/1 -> Switch/2
  Unit Delay/1 -> Sum2/2
  Constant1/1 -> Switch/3
  Min2/1 -> Switch/1
  Constant/1 -> Sum2/1
  Constant2/1 -> Relational Operator/2, Min2/2
  Sum2/1 -> Min2/1, Relational Operator/1

== system controls_element_lib/acChecks_A/Assert Timer4 ==
  in : Inport
  Constant : Constant  Value=T_STEP
  Constant1 : Constant  Value=0
  Constant2 : Constant  Value=TIMEOUT
  Min2 : MinMax  Inputs=2
  Relational Operator : RelationalOperator  Operator=>  OutDataTypeStr=boolean  RndMeth=Simplest
  Sum2 : Sum  Inputs=|++
  Switch : Switch  Criteria=u2 > Threshold
  Unit Delay : UnitDelay  SampleTime=T_STEP  HasFrameUpgradeWarning=on
  out : Outport
  wires:
  Sum2/1 -> Relational Operator/1, Min2/1
  Constant2/1 -> Min2/2, Relational Operator/2
  Constant/1 -> Sum2/1
  Min2/1 -> Switch/1
  Constant1/1 -> Switch/3
  Unit Delay/1 -> Sum2/2
  in/1 -> Switch/2
  Switch/1 -> Unit Delay/1
  Relational Operator/1 -> out/1

== system controls_element_lib/acChecks_A/Assert Timer5 ==
  in : Inport
  Constant : Constant  Value=T_STEP
  Constant1 : Constant  Value=0
  Constant2 : Constant  Value=TIMEOUT
  Min2 : MinMax  Inputs=2
  Relational Operator : RelationalOperator  Operator=>  OutDataTypeStr=boolean  RndMeth=Simplest
  Sum2 : Sum  Inputs=|++
  Switch : Switch  Criteria=u2 > Threshold
  Unit Delay : UnitDelay  SampleTime=T_STEP  HasFrameUpgradeWarning=on
  out : Outport
  wires:
  Sum2/1 -> Relational Operator/1, Min2/1
  Constant2/1 -> Min2/2, Relational Operator/2
  Constant/1 -> Sum2/1
  Min2/1 -> Switch/1
  Constant1/1 -> Switch/3
  Unit Delay/1 -> Sum2/2
  in/1 -> Switch/2
  Switch/1 -> Unit Delay/1
  Relational Operator/1 -> out/1

== system controls_element_lib/acChecks_A/Assert Timer6 ==
  in : Inport
  Constant : Constant  Value=T_STEP
  Constant1 : Constant  Value=0
  Constant2 : Constant  Value=TIMEOUT
  Min2 : MinMax  Inputs=2
  Relational Operator : RelationalOperator  Operator=>  OutDataTypeStr=boolean  RndMeth=Simplest
  Sum2 : Sum  Inputs=|++
  Switch : Switch  Criteria=u2 > Threshold
  Unit Delay : UnitDelay  SampleTime=T_STEP  HasFrameUpgradeWarning=on
  out : Outport
  wires:
  Relational Operator/1 -> out/1
  Switch/1 -> Unit Delay/1
  in/1 -> Switch/2
  Unit Delay/1 -> Sum2/2
  Constant1/1 -> Switch/3
  Min2/1 -> Switch/1
  Constant/1 -> Sum2/1
  Constant2/1 -> Relational Operator/2, Min2/2
  Sum2/1 -> Min2/1, Relational Operator/1

== system controls_element_lib/acChecks_A/Assert Timer7 ==
  in : Inport
  Constant : Constant  Value=T_STEP
  Constant1 : Constant  Value=0
  Constant2 : Constant  Value=TIMEOUT
  Min2 : MinMax  Inputs=2
  Relational Operator : RelationalOperator  Operator=>  OutDataTypeStr=boolean  RndMeth=Simplest
  Sum2 : Sum  Inputs=|++
  Switch : Switch  Criteria=u2 > Threshold
  Unit Delay : UnitDelay  SampleTime=T_STEP  HasFrameUpgradeWarning=on
  out : Outport
  wires:
  Sum2/1 -> Relational Operator/1, Min2/1
  Constant2/1 -> Min2/2, Relational Operator/2
  Constant/1 -> Sum2/1
  Min2/1 -> Switch/1
  Constant1/1 -> Switch/3
  Unit Delay/1 -> Sum2/2
  in/1 -> Switch/2
  Switch/1 -> Unit Delay/1
  Relational Operator/1 -> out/1

== system controls_element_lib/acChecks_A/Assert Timer8 ==
  in : Inport
  Constant : Constant  Value=T_STEP
  Constant1 : Constant  Value=0
  Constant2 : Constant  Value=TIMEOUT
  Min2 : MinMax  Inputs=2
  Relational Operator : RelationalOperator  Operator=>  OutDataTypeStr=boolean  RndMeth=Simplest
  Sum2 : Sum  Inputs=|++
  Switch : Switch  Criteria=u2 > Threshold
  Unit Delay : UnitDelay  SampleTime=T_STEP  HasFrameUpgradeWarning=on
  out : Outport
  wires:
  Relational Operator/1 -> out/1
  Switch/1 -> Unit Delay/1
  in/1 -> Switch/2
  Unit Delay/1 -> Sum2/2
  Constant1/1 -> Switch/3
  Min2/1 -> Switch/1
  Constant/1 -> Sum2/1
  Constant2/1 -> Relational Operator/2, Min2/2
  Sum2/1 -> Min2/1, Relational Operator/1

== system controls_element_lib/acChecks_A/Clear Timer1 ==
  in : Inport
  Constant : Constant  Value=T_STEP
  Constant1 : Constant  Value=0
  Constant2 : Constant  Value=TIMEOUT
  Min2 : MinMax  Function=max  Inputs=2
  Relational Operator : RelationalOperator  Operator=>  OutDataTypeStr=boolean  RndMeth=Simplest
  Sum2 : Sum  Inputs=|-+
  Switch : Switch  Criteria=u2 > Threshold
  Unit Delay : UnitDelay  InitialCondition=TIMER_INIT  SampleTime=T_STEP  HasFrameUpgradeWarning=on
  out : Outport
  wires:
  Constant2/1 -> Switch/1
  Sum2/1 -> Relational Operator/1, Min2/1
  Constant/1 -> Sum2/1
  Min2/1 -> Switch/3
  Constant1/1 -> Min2/2, Relational Operator/2
  Unit Delay/1 -> Sum2/2
  in/1 -> Switch/2
  Switch/1 -> Unit Delay/1
  Relational Operator/1 -> out/1

== system controls_element_lib/acChecks_A/Clear Timer10 ==
  in : Inport
  Constant : Constant  Value=T_STEP
  Constant1 : Constant  Value=0
  Constant2 : Constant  Value=TIMEOUT
  Min2 : MinMax  Function=max  Inputs=2
  Relational Operator : RelationalOperator  Operator=>  OutDataTypeStr=boolean  RndMeth=Simplest
  Sum2 : Sum  Inputs=|-+
  Switch : Switch  Criteria=u2 > Threshold
  Unit Delay : UnitDelay  InitialCondition=TIMER_INIT  SampleTime=T_STEP  HasFrameUpgradeWarning=on
  out : Outport
  wires:
  Constant2/1 -> Switch/1
  Sum2/1 -> Relational Operator/1, Min2/1
  Constant/1 -> Sum2/1
  Min2/1 -> Switch/3
  Constant1/1 -> Min2/2, Relational Operator/2
  Unit Delay/1 -> Sum2/2
  in/1 -> Switch/2
  Switch/1 -> Unit Delay/1
  Relational Operator/1 -> out/1

== system controls_element_lib/acChecks_A/Clear Timer11 ==
  in : Inport
  Constant : Constant  Value=T_STEP
  Constant1 : Constant  Value=0
  Constant2 : Constant  Value=TIMEOUT
  Min2 : MinMax  Function=max  Inputs=2
  Relational Operator : RelationalOperator  Operator=>  OutDataTypeStr=boolean  RndMeth=Simplest
  Sum2 : Sum  Inputs=|-+
  Switch : Switch  Criteria=u2 > Threshold
  Unit Delay : UnitDelay  InitialCondition=TIMER_INIT  SampleTime=T_STEP  HasFrameUpgradeWarning=on
  out : Outport
  wires:
  Relational Operator/1 -> out/1
  Switch/1 -> Unit Delay/1
  in/1 -> Switch/2
  Unit Delay/1 -> Sum2/2
  Constant1/1 -> Relational Operator/2, Min2/2
  Min2/1 -> Switch/3
  Constant/1 -> Sum2/1
  Sum2/1 -> Min2/1, Relational Operator/1
  Constant2/1 -> Switch/1

== system controls_element_lib/acChecks_A/Clear Timer2 ==
  in : Inport
  Constant : Constant  Value=T_STEP
  Constant1 : Constant  Value=0
  Constant2 : Constant  Value=TIMEOUT
  Min2 : MinMax  Function=max  Inputs=2
  Relational Operator : RelationalOperator  Operator=>  OutDataTypeStr=boolean  RndMeth=Simplest
  Sum2 : Sum  Inputs=|-+
  Switch : Switch  Criteria=u2 > Threshold
  Unit Delay : UnitDelay  InitialCondition=TIMER_INIT  SampleTime=T_STEP  HasFrameUpgradeWarning=on
  out : Outport
  wires:
  Relational Operator/1 -> out/1
  Switch/1 -> Unit Delay/1
  in/1 -> Switch/2
  Unit Delay/1 -> Sum2/2
  Constant1/1 -> Relational Operator/2, Min2/2
  Min2/1 -> Switch/3
  Constant/1 -> Sum2/1
  Sum2/1 -> Min2/1, Relational Operator/1
  Constant2/1 -> Switch/1

== system controls_element_lib/acChecks_A/Clear Timer3 ==
  in : Inport
  Constant : Constant  Value=T_STEP
  Constant1 : Constant  Value=0
  Constant2 : Constant  Value=TIMEOUT
  Min2 : MinMax  Function=max  Inputs=2
  Relational Operator : RelationalOperator  Operator=>  OutDataTypeStr=boolean  RndMeth=Simplest
  Sum2 : Sum  Inputs=|-+
  Switch : Switch  Criteria=u2 > Threshold
  Unit Delay : UnitDelay  InitialCondition=TIMER_INIT  SampleTime=T_STEP  HasFrameUpgradeWarning=on
  out : Outport
  wires:
  Constant2/1 -> Switch/1
  Sum2/1 -> Relational Operator/1, Min2/1
  Constant/1 -> Sum2/1
  Min2/1 -> Switch/3
  Constant1/1 -> Min2/2, Relational Operator/2
  Unit Delay/1 -> Sum2/2
  in/1 -> Switch/2
  Switch/1 -> Unit Delay/1
  Relational Operator/1 -> out/1

== system controls_element_lib/acChecks_A/Clear Timer4 ==
  in : Inport
  Constant : Constant  Value=T_STEP
  Constant1 : Constant  Value=0
  Constant2 : Constant  Value=TIMEOUT
  Min2 : MinMax  Function=max  Inputs=2
  Relational Operator : RelationalOperator  Operator=>  OutDataTypeStr=boolean  RndMeth=Simplest
  Sum2 : Sum  Inputs=|-+
  Switch : Switch  Criteria=u2 > Threshold
  Unit Delay : UnitDelay  InitialCondition=TIMER_INIT  SampleTime=T_STEP  HasFrameUpgradeWarning=on
  out : Outport
  wires:
  Relational Operator/1 -> out/1
  Switch/1 -> Unit Delay/1
  in/1 -> Switch/2
  Unit Delay/1 -> Sum2/2
  Constant1/1 -> Relational Operator/2, Min2/2
  Min2/1 -> Switch/3
  Constant/1 -> Sum2/1
  Sum2/1 -> Min2/1, Relational Operator/1
  Constant2/1 -> Switch/1

== system controls_element_lib/acChecks_A/Clear Timer5 ==
  in : Inport
  Constant : Constant  Value=T_STEP
  Constant1 : Constant  Value=0
  Constant2 : Constant  Value=TIMEOUT
  Min2 : MinMax  Function=max  Inputs=2
  Relational Operator : RelationalOperator  Operator=>  OutDataTypeStr=boolean  RndMeth=Simplest
  Sum2 : Sum  Inputs=|-+
  Switch : Switch  Criteria=u2 > Threshold
  Unit Delay : UnitDelay  InitialCondition=TIMER_INIT  SampleTime=T_STEP  HasFrameUpgradeWarning=on
  out : Outport
  wires:
  Relational Operator/1 -> out/1
  Switch/1 -> Unit Delay/1
  in/1 -> Switch/2
  Unit Delay/1 -> Sum2/2
  Constant1/1 -> Relational Operator/2, Min2/2
  Min2/1 -> Switch/3
  Constant/1 -> Sum2/1
  Sum2/1 -> Min2/1, Relational Operator/1
  Constant2/1 -> Switch/1

== system controls_element_lib/acChecks_A/Clear Timer6 ==
  in : Inport
  Constant : Constant  Value=T_STEP
  Constant1 : Constant  Value=0
  Constant2 : Constant  Value=TIMEOUT
  Min2 : MinMax  Function=max  Inputs=2
  Relational Operator : RelationalOperator  Operator=>  OutDataTypeStr=boolean  RndMeth=Simplest
  Sum2 : Sum  Inputs=|-+
  Switch : Switch  Criteria=u2 > Threshold
  Unit Delay : UnitDelay  InitialCondition=TIMER_INIT  SampleTime=T_STEP  HasFrameUpgradeWarning=on
  out : Outport
  wires:
  Constant2/1 -> Switch/1
  Sum2/1 -> Relational Operator/1, Min2/1
  Constant/1 -> Sum2/1
  Min2/1 -> Switch/3
  Constant1/1 -> Min2/2, Relational Operator/2
  Unit Delay/1 -> Sum2/2
  in/1 -> Switch/2
  Switch/1 -> Unit Delay/1
  Relational Operator/1 -> out/1

== system controls_element_lib/acChecks_A/Clear Timer7 ==
  in : Inport
  Constant : Constant  Value=T_STEP
  Constant1 : Constant  Value=0
  Constant2 : Constant  Value=TIMEOUT
  Min2 : MinMax  Function=max  Inputs=2
  Relational Operator : RelationalOperator  Operator=>  OutDataTypeStr=boolean  RndMeth=Simplest
  Sum2 : Sum  Inputs=|-+
  Switch : Switch  Criteria=u2 > Threshold
  Unit Delay : UnitDelay  InitialCondition=TIMER_INIT  SampleTime=T_STEP  HasFrameUpgradeWarning=on
  out : Outport
  wires:
  Relational Operator/1 -> out/1
  Switch/1 -> Unit Delay/1
  in/1 -> Switch/2
  Unit Delay/1 -> Sum2/2
  Constant1/1 -> Relational Operator/2, Min2/2
  Min2/1 -> Switch/3
  Constant/1 -> Sum2/1
  Sum2/1 -> Min2/1, Relational Operator/1
  Constant2/1 -> Switch/1

== system controls_element_lib/acChecks_A/Clear Timer8 ==
  in : Inport
  Constant : Constant  Value=T_STEP
  Constant1 : Constant  Value=0
  Constant2 : Constant  Value=TIMEOUT
  Min2 : MinMax  Function=max  Inputs=2
  Relational Operator : RelationalOperator  Operator=>  OutDataTypeStr=boolean  RndMeth=Simplest
  Sum2 : Sum  Inputs=|-+
  Switch : Switch  Criteria=u2 > Threshold
  Unit Delay : UnitDelay  InitialCondition=TIMER_INIT  SampleTime=T_STEP  HasFrameUpgradeWarning=on
  out : Outport
  wires:
  Constant2/1 -> Switch/1
  Sum2/1 -> Relational Operator/1, Min2/1
  Constant/1 -> Sum2/1
  Min2/1 -> Switch/3
  Constant1/1 -> Min2/2, Relational Operator/2
  Unit Delay/1 -> Sum2/2
  in/1 -> Switch/2
  Switch/1 -> Unit Delay/1
  Relational Operator/1 -> out/1

== system controls_element_lib/acChecks_A/Clear Timer9 ==
  in : Inport
  Constant : Constant  Value=T_STEP
  Constant1 : Constant  Value=0
  Constant2 : Constant  Value=TIMEOUT
  Min2 : MinMax  Function=max  Inputs=2
  Relational Operator : RelationalOperator  Operator=>  OutDataTypeStr=boolean  RndMeth=Simplest
  Sum2 : Sum  Inputs=|-+
  Switch : Switch  Criteria=u2 > Threshold
  Unit Delay : UnitDelay  InitialCondition=TIMER_INIT  SampleTime=T_STEP  HasFrameUpgradeWarning=on
  out : Outport
  wires:
  Relational Operator/1 -> out/1
  Switch/1 -> Unit Delay/1
  in/1 -> Switch/2
  Unit Delay/1 -> Sum2/2
  Constant1/1 -> Relational Operator/2, Min2/2
  Min2/1 -> Switch/3
  Constant/1 -> Sum2/1
  Sum2/1 -> Min2/1, Relational Operator/1
  Constant2/1 -> Switch/1

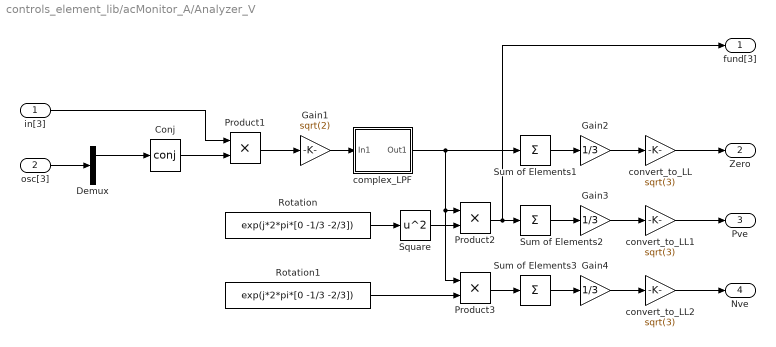
== system controls_element_lib/acMonitor_A/Analyzer_V ==
  in[3] : Inport
  osc[3] : Inport  Port=2
  Conj : Math  Operator=conj  SaturateOnIntegerOverflow=on
  Demux : Demux  Outputs=3
  Gain1 : Gain  Gain=sqrt(2)
  Gain2 : Gain  Gain=1/3
  Gain3 : Gain  Gain=1/3
  Gain4 : Gain  Gain=1/3
  Product1 : Product
  Product2 : Product
  Product3 : Product
  Rotation : Constant  Value=exp(j*2*pi*[0 -1/3 -2/3])
  Rotation1 : Constant  Value=exp(j*2*pi*[0 -1/3 -2/3])
  Square : Math  Operator=square  SaturateOnIntegerOverflow=on
  Sum of Elements1 : Sum  Inputs=+
  Sum of Elements2 : Sum  Inputs=+
  Sum of Elements3 : Sum  Inputs=+
  complex_LPF : Subsystem  mask{tau=0.05}
      mask prompts: tau "Time constant"
  convert_to_LL : Gain  Gain=sqrt(3)
  convert_to_LL1 : Gain  Gain=sqrt(3)
  convert_to_LL2 : Gain  Gain=sqrt(3)
  fund[3] : Outport
  Zero : Outport  Port=2
  Pve : Outport  Port=3
  Nve : Outport  Port=4
  wires:
  in[3]/1 -> Product1/1
  Gain2/1 -> convert_to_LL/1
  Gain3/1 -> convert_to_LL1/1
  osc[3]/1 -> Demux/1
  Sum of Elements3/1 -> Gain4/1
  Square/1 -> Product2/2
  Sum of Elements1/1 -> Gain2/1
  Conj/1 -> Product1/2
  Sum of Elements2/1 -> Gain3/1
  Rotation1/1 -> Product3/2
  Rotation/1 -> Square/1
  Demux/1 -> Conj/1
  Gain1/1 -> complex_LPF/1(In1)
  Product3/1 -> Sum of Elements3/1
  Product1/1 -> Gain1/1
  complex_LPF/1(Out1) -> Sum of Elements1/1, Product2/1, Product3/1
  Product2/1 -> Sum of Elements2/1, fund[3]/1
  Gain4/1 -> convert_to_LL2/1
  convert_to_LL/1 -> Zero/1
  convert_to_LL1/1 -> Pve/1
  convert_to_LL2/1 -> Nve/1

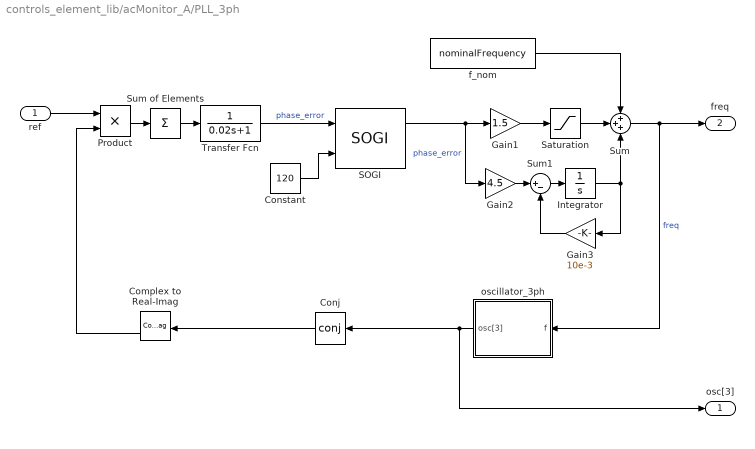
== system controls_element_lib/acMonitor_A/PLL_3ph ==
  ref : Inport
  Complex to Real-Imag : ComplexToRealImag
  Conj : Math  Operator=conj  SaturateOnIntegerOverflow=on
  Constant : Constant  Value=120
  Gain1 : Gain  Gain=1.5
  Gain2 : Gain  Gain=4.5
  Gain3 : Gain  Gain=10e-3
  Integrator : Integrator  LimitOutput=on  UpperSaturationLimit=5  LowerSaturationLimit=-5
  Product : Product
  SOGI : $bdroot/dcVoltageRegulator_A/SOGI  SystemSampleTime=-1  EmptyChoice=off  PassThrough=off  PassThroughVariantControl=(default)  EmptyChoiceVariantControl=(default)  Latency=0  AutoFrameSizeCalculation=off
  Saturation : Saturate  UpperLimit=5  LowerLimit=-5
  Sum : Sum  Inputs=+++
  Sum of Elements : Sum  Inputs=+
  Sum1 : Sum  Inputs=|+-
  Transfer Fcn : TransferFcn  Denominator=[0.02 1]
  f_nom : Constant  Value=nominalFrequency
  oscillator_3ph : Subsystem
  osc[3] : Outport
  freq : Outport  Port=2
  wires:
  Gain1/1 -> Saturation/1
  Conj/1 -> Complex to Real-Imag/1
  ref/1 -> Product/1
  Integrator/1 -> Sum/3, Gain3/1
  Sum1/1 -> Integrator/1
  Complex to Real-Imag/2 -> Product/2
  Gain2/1 -> Sum1/1
  oscillator_3ph/1(osc[3]) -> osc[3]/1, Conj/1
  Sum/1 -> oscillator_3ph/1(f), freq/1  "freq"
  Product/1 -> Sum of Elements/1
  Saturation/1 -> Sum/2
  SOGI/1 -> Gain2/1, Gain1/1  "phase_error"
  Sum of Elements/1 -> Transfer Fcn/1
  Gain3/1 -> Sum1/2
  f_nom/1 -> Sum/1
  Transfer Fcn/1 -> SOGI/1  "phase_error"
  Constant/1 -> SOGI/2

== system controls_element_lib/acMonitor_A/RMS_Analyzer ==
  in : Inport
  Gain : Gain  Gain=2 * pi * 10
  Integrator : Integrator  InitialCondition=0.01
  Sqrt : Sqrt  SaturateOnIntegerOverflow=on
  Square : Math  Operator=square  SaturateOnIntegerOverflow=on
  Sum : Sum  Inputs=|+-
  RMS : Outport
  wires:
  Sqrt/1 -> RMS/1
  Integrator/1 -> Sqrt/1, Sum/2
  Sum/1 -> Gain/1
  Gain/1 -> Integrator/1
  in/1 -> Square/1
  Square/1 -> Sum/1
